simulink model "simple_constant_deceleration"  (R2024a)
settings: Solver=ode1  StartTime=0.0  StopTime=10  FixedStep=0.001  RelTol=1e-3
PostLoadFcn:
  | , if any(exist('dsrtsu_mdlpostloadfcn', 'file') == [2, 3, 6]), try dsrtsu_mdlpostloadfcn('Execute', bdroot); catch fprintf('Error in PostLoadFcn (dsrtsu_mdlpostloadfcn) for model "%s":\n %s\n', bdroot, lasterr); end, end,
InitFcn:
  | , if any(exist('rtifpga_mdlclblib', 'file') ~= 0), rtifpga_mdlclblib('Init', bdroot); end,
values from neighbouring files (symbols this model uses):
  a = 1.2    [init_parameters.m]
  Ap = [0, 1, 0, 0 ... (first row only)    [init_parameters.m]
  As = Ap    [init_parameters.m]
  b = 1.6    [init_parameters.m]
  Bp = [0 ... (first row only)    [init_parameters.m]
  Bs = [0, 0, 0 ... (first row only)    [init_parameters.m]
  c_max = 4000    [init_parameters.m]
  c_min = 500    [init_parameters.m]
  Cp = eye(4)    [init_parameters.m]
  Cs = Cp    [init_parameters.m]
  Dp = zeros(4, 1)    [init_parameters.m]
  Ds = zeros(4, 3)    [init_parameters.m]
  K = lqr(As, B_control, Q, R)    [init_parameters.m]
Description:
  | Standard RTI1401 template.
  | Supported MATLAB version:  R2024a.
settings Model: Tag=RTI1401  DSRTSU_INTERNAL_RTI_VER=640  DSRTSU_INTERNAL_RTI_TYPE=rti1401  RTICANMMDATA=struct('GeneralSetupData',struct('modelroot','C:\Users\VM-User\Desktop\MigrationScripts','generalsettings',struct('filesettings',struct('destfolder',struct('Name','RTICANMM_FILES','Check',1),'buildfolder',struct('Name','.','Check',1),'AbsDestfolder',struct('Name','C:\Users\VM-User\Desktop\MigrationScripts\RTICANMM_FILES'),'AbsBuildfolder',struct('Name','C:\Users\VM-User\Desktop\MigrationScripts'))),'options',struct('addpaths',1,'rmpaths',1,'addtrcexclusion',true,'cannavigator',struct('checkmonitoring',0),'show_usrtrc',0,'use_usrtrc',0),'advanced',struct('options',ones(1,100)),'MPSetup',{{}},'RTI',struct('Type','RTI1401','Ver','7.17','Date','02-Nov-2021'),'modelname','','block','untitled'))  DSRTSU_INTERNAL_RTIFPGA=210  DSRTSU_INTERNAL_RTISTBM_VER=24.1  Creator=ivanv  LastModifiedBy=ivanv
settings SolverCC: AlgebraicLoopSolver=TrustRegion
settings DataIOCC: ReturnWorkspaceOutputs=off
settings OptimizationCC: BlockReduction=off  OptimizeBlockIOStorage=off  BufferReuse=off  ReuseModelBlockBuffer=off  GlobalBufferReuse=off  ExpressionFolding=off  LocalBlockOutputs=off  OptimizeDataStoreBuffers=off  BusAssignmentInplaceUpdate=off
settings DebuggingCC: UnconnectedInputMsg=warning  UnconnectedOutputMsg=warning  UnconnectedLineMsg=warning  PregeneratedLibrarySubsystemCodeDiagnostic=none  ArithmeticOperatorsInVariantConditions=warning
settings HardwareCC: ProdBitPerPointer=32  ProdBitPerSizeT=32  ProdBitPerPtrDiffT=32  ProdLargestAtomicInteger=Integer  ProdEndianess=BigEndian  ProdWordSize=32  ProdLongLongMode=on  ProdHWDeviceType=Custom Processor->Custom  TargetIntDivRoundTo=Zero  TargetEndianess=BigEndian  TargetHWDeviceType=Custom Processor->Custom
settings ModelReferenceCC: EnableRefExpFcnMdlSchedulingChecks=on  EnableParallelModelReferenceBuilds=on  ParallelModelReferenceMATLABWorkerInit=Load Top Model
settings SFSimCC: SimUseLocalCustomCode=off  MATLABDynamicMemAlloc=off  CustomCodeUndefinedFunction=UseInterfaceOnly
settings RTWCC: Description=dSPACE DS1401 Hardware Platform  SystemTargetFile=rti1401.tlc  MakeCommand=make_rti  TemplateMakefile=rti1401.tmf  RTWUseLocalCustomCode=off  GPUComputeCapability=3.5  DLArmComputeVersion=19.05
settings CodeAppCC: StateflowObjectComments=on
settings STFCustomTargetCC: TargetLangStandard=C89/C90 (ANSI)  ParMdlRefBuildCompliant=on  MatFileLogging=on  GRTInterface=off  UseToolchainInfoCompliant=off  SystemTargetFile=rti1401.tlc
settings GRTTargetCC: TargetLangStandard=C89/C90 (ANSI)  CompOptLevelCompliant=off  ConcurrentExecutionCompliant=off  CombineOutputUpdateFcns=off  CPPClassGenCompliant=off  UseToolchainInfoCompliant=off
settings ConfigComp: CovMetricSettings=dswe

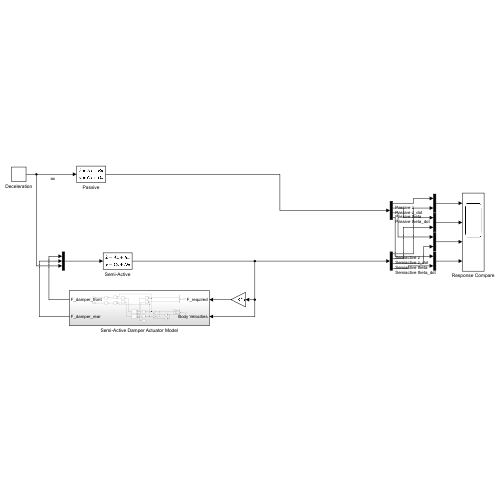
[thumbnail: Simulink's stored preview of the top-level diagram]
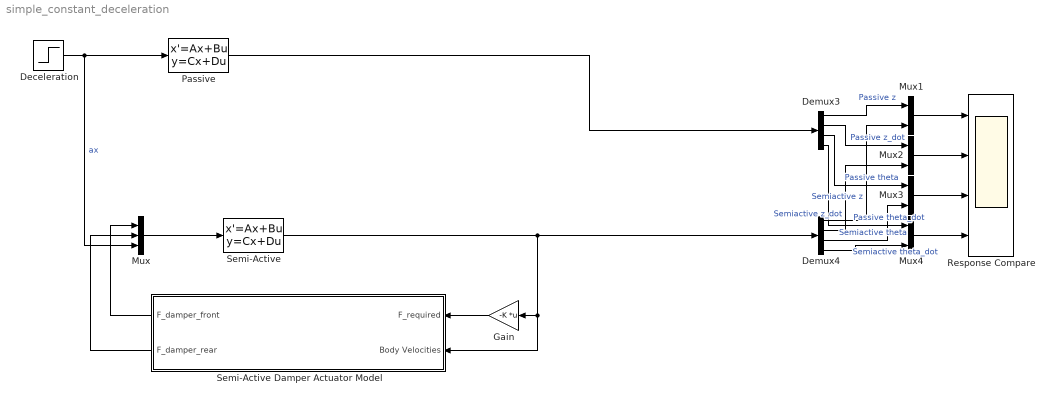
== system simple_constant_deceleration ==
  Deceleration : Step  After=8  SampleTime=0
  Demux3 : Demux
  Demux4 : Demux
  Gain : Gain  Gain=-K  Multiplication=Matrix(K*u)
  Mux : Mux  Inputs=3
  Mux{1..4} (4 alike) : Mux  Inputs=2
  Passive : StateSpace  A=Ap  B=Bp  C=Cp  D=Dp  InitialCondition=0
  Response Compare : Scope  NumInputPorts=4
  Semi-Active : StateSpace  A=As  B=Bs  C=Cs  D=Ds  InitialCondition=0
  Semi-Active Damper Actuator Model : Subsystem
  wires:
  Deceleration/1 -> Mux/3, Passive/1  "ax"
  Passive/1 -> Demux3/1
  Mux/1 -> Semi-Active/1
  Semi-Active/1 -> Demux4/1, Semi-Active Damper Actuator Model/2(Body Velocities), Gain/1
  Mux1/1 -> Response Compare/1
  Mux2/1 -> Response Compare/2
  Mux3/1 -> Response Compare/3
  Mux4/1 -> Response Compare/4
  Demux3/1 -> Mux1/1  "Passive z"
  Demux4/1 -> Mux1/2  "Semiactive z"
  Demux3/2 -> Mux2/1  "Passive z_dot"
  Demux4/2 -> Mux2/2  "Semiactive z_dot"
  Demux3/3 -> Mux3/1  "Passive theta"
  Demux4/3 -> Mux3/2  "Semiactive theta"
  Demux3/4 -> Mux4/1  "Passive theta_dot"
  Demux4/4 -> Mux4/2  "Semiactive theta_dot"
  Gain/1 -> Semi-Active Damper Actuator Model/1(F_required)
  Semi-Active Damper Actuator Model/1(F_damper_front) -> Mux/1
  Semi-Active Damper Actuator Model/2(F_damper_rear) -> Mux/2

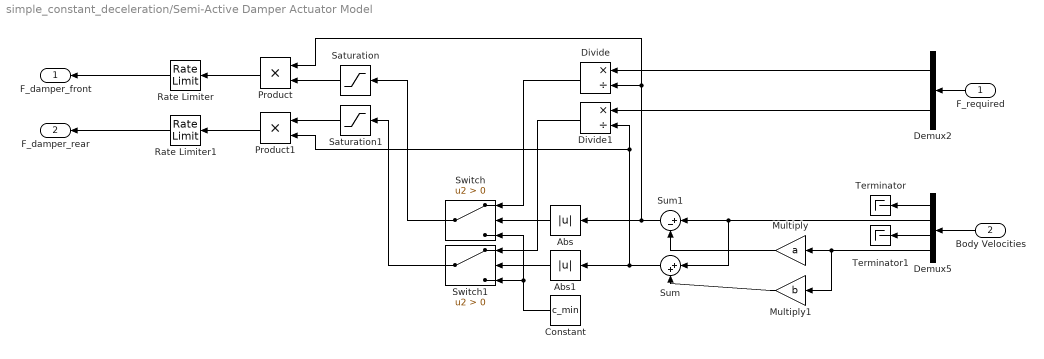
== system simple_constant_deceleration/Semi-Active Damper Actuator Model ==
  F_required : Inport
  Body Velocities : Inport  Port=2
  Abs : Abs  SaturateOnIntegerOverflow=off
  Abs1 : Abs  SaturateOnIntegerOverflow=off
  Constant : Constant  Value=c_min
  Demux2 : Demux  Outputs=2
  Demux5 : Demux
  Divide : Product  Inputs=*/
  Divide1 : Product  Inputs=*/
  Multiply : Gain  Gain=a
  Multiply1 : Gain  Gain=b
  Product : Product
  Product1 : Product
  Rate Limiter : RateLimiter  RisingSlewLimit=175000  FallingSlewLimit=-175000  SampleTimeMode=inherited
  Rate Limiter1 : RateLimiter  RisingSlewLimit=175000  FallingSlewLimit=-175000  SampleTimeMode=inherited
  Saturation : Saturate  UpperLimit=c_max  LowerLimit=c_min
  Saturation1 : Saturate  UpperLimit=c_max  LowerLimit=c_min
  Sum : Sum  Inputs=|++
  Sum1 : Sum  Inputs=|+-
  Switch : Switch  Criteria=u2 > Threshold  SaturateOnIntegerOverflow=off  InputSameDT=off
  Switch1 : Switch  Criteria=u2 > Threshold  SaturateOnIntegerOverflow=off  InputSameDT=off
  Terminator : Terminator
  Terminator1 : Terminator
  F_damper_front : Outport
  F_damper_rear : Outport  Port=2
  wires:
  Constant/1 -> Switch/3, Switch1/3
  Demux5/1 -> Terminator/1
  Demux5/4 -> Multiply1/1, Multiply/1
  Sum1/1 -> Abs/1, Product/1, Divide/2
  Demux2/1 -> Divide/1
  Body Velocities/1 -> Demux5/1
  Saturation/1 -> Product/2
  Demux5/2 -> Sum1/1, Sum/1
  Abs/1 -> Switch/2
  Product/1 -> Rate Limiter/1
  Switch1/1 -> Saturation1/1
  Divide/1 -> Switch/1
  Switch/1 -> Saturation/1
  Sum/1 -> Abs1/1, Product1/2, Divide1/2
  Demux2/2 -> Divide1/1
  Rate Limiter1/1 -> F_damper_rear/1
  Multiply1/1 -> Sum/2
  F_required/1 -> Demux2/1
  Abs1/1 -> Switch1/2
  Saturation1/1 -> Product1/1
  Multiply/1 -> Sum1/2
  Demux5/3 -> Terminator1/1
  Product1/1 -> Rate Limiter1/1
  Divide1/1 -> Switch1/1
  Rate Limiter/1 -> F_damper_front/1
